simulink model "furuta_hybrid_model"  (R2026b)
settings: Solver=ode23t  StopTime=0.25  MaxStep=5.0000000000000002e-05  RelTol=1e-5  AbsTol=1e-8
model workspace (MAT data in the model file):
  cfg.sampleTime = 0.005
  cfg.energyGain = 100
  cfg.energyOffset = 0.04
  cfg.armCenterGain = 4
  cfg.armDampingGain = 3
  cfg.accelerationLimit = 25
  cfg.kickAcceleration = 3
  cfg.kickRate = 0.03
  cfg.signSlope = 8
  cfg.voltageLimit = 12
  cfg.captureAngle = 0.314159265359
  cfg.captureRate = 3
  cfg.captureArmRate = 3
  cfg.captureVoltage = 10
  cfg.releaseAngle = 0.610865238198
  cfg.releaseRate = 6
  cfg.armLimit = 3.14159265359
  cfg.speedLimit = 20
  disableTime = 100
  drive.voltageLimit = 12
  drive.resistance = 6.00258223899
  drive.backEmfOutput = 0.535780000531
  drive.torqueConstantOutput = 0.15
  drive.gearRatioSigned = -35.0048
  drive.gearRatio = 35.0048
  drive.motorShaftDamping = 4.08e-09
  drive.armatureInductance = 1.2003374e-05
  drive.gearEfficiency = 0.74571885855
  drive.speedGain = 1.74515107433
  drive.timeConstant = 0.200035574902
  drive.viscousDamping = 4.999370974e-06
  drive.reflectedInertia = 0.0028643583489
  drive.backEmfMotor = 0.0153059009202
  drive.torqueConstantMotor = 0.0057463031303
  drive.bridgeDrop = 2.55
  drive.pwmFrequency = 1000
  enableTime = 0
  furutaCoverImages.system = [242 242 242 242 242 242 242 242 242 242 242 242 ... (162435 elements, 221x245x3)]
  furutaCoverImages.bridge = [255 255 255 255 255 255 255 255 255 255 255 255 ... (561330 elements, 378x495x3)]
  furutaCoverImages.motor = [255 255 255 255 255 255 255 255 255 255 255 255 ... (578340 elements, 378x510x3)]
  furutaCoverImages.plant = [242 242 242 242 242 242 242 242 242 242 242 242 ... (57240 elements, 106x180x3)]
  initialState = [0; 3.14159265359; 0; 0]
  p.source = 'Revised Inventor Assembly1.iam with two fixed aluminum profiles'
  p.units = 'm, kg, kg*m^2, rad, N*m'
  p.parts(1).name = 'Motor_1'
  p.parts(1).source = 'cad\originals\inventor-package\modern control\modern control\Motor.ipt'
  p.parts(1).group = 'base'
  p.parts(1).rotation = [0.999875892244  0.0157543679293  8.87132397872e-16; 0.0157543679293  -0.999875892244  6.0713824632e-16; 8.96587377177e-16  -5.93086685557e-16  -1]
  p.parts(1).translation = [-7.8496237288e-17; 0; 0.0574]
  p.parts(1).mass = 0.117533764135
  p.parts(1).com = [-2.51629547723e-06; 7.77686868846e-05; 0.0334585043492]
  p.parts(1).inertia = [4.21856071427e-05  1.61868677081e-09  -2.41973308628e-09; 1.61868677081e-09  4.21259722545e-05  3.40164241998e-07; -2.41973308628e-09  3.40164241998e-07  9.42409412023e-06]
  p.parts(1).mesh = 'Motor_1.stl'
  p.parts(2).name = 'motor_holder_1'
  p.parts(2).source = 'cad\originals\inventor-package\modern control\modern control\motor holder.ipt'
  p.parts(2).group = 'base'
  p.parts(2).rotation = [-0.999993667555  -0.0035587708406  -8.83740457218e-16; 0.0035587708406  -0.999993667555  -6.03187801199e-16; -8.81588253822e-16  -6.06329011316e-16  1]
  p.parts(2).translation = [7.47341876526e-05; 0.0209998670187; 0.0183]
  p.parts(2).mass = 0.00752339947436
  p.parts(2).com = [1.89560478822e-14; 0.00840615914464; -0.00851588759587]
  p.parts(2).inertia = [1.56089117939e-06  -1.79636877134e-18  1.13827387038e-18; -1.79636877134e-18  1.27680196487e-06  4.44884161923e-07; 1.13827387038e-18  4.44884161923e-07  1.17145571104e-06]
  p.parts(2).mesh = 'motor_holder_1.stl'
  p.parts(3).name = 'Assembly2_1'
  p.parts(3).source = 'cad\originals\inventor-package\modern control\modern control\Assembly2\Assembly2.iam'
  p.parts(3).group = 'arm'
  p.parts(3).rotation = [-9.59608079282e-17  1.42983226155e-16  -1; 1.46439076445e-15  1  2.58616733772e-16; 1  -1.46439076445e-15  -9.59608079283e-17]
  p.parts(3).translation = [-0.00424079872686; -0.00199057601285; -0.0717771991128]
  p.parts(3).mass = 0.0256607587457
  p.parts(3).com = [0.0543345548641; 0.00199067178848; -0.00669149901998]
  p.parts(3).inertia = [3.76240629517e-06  -1.16658650356e-10  -1.25869727666e-06; -1.16658650356e-10  5.41849992051e-06  3.32034498219e-10; -1.25869727666e-06  3.32034498219e-10  5.39265534854e-06]
  p.parts(3).mesh = 'Assembly2_1.stl'
  p.parts(4).name = 'ROTERY_ENCODER_step_2'
  p.parts(4).source = 'cad\originals\inventor-package\modern control\modern control\ROTERY ENCODER.step.ipt'
  p.parts(4).group = 'arm'
  p.parts(4).rotation = [5.71932904618e-15  1  2.07325677924e-15; -0.795351383406  -6.03439045467e-16  -0.606148642591; -0.606148642591  4.20921426938e-17  0.795351383406]
  p.parts(4).translation = [-0.018; -2.55922809462e-17; -0.039]
  p.parts(4).mass = 0.362581648921
  p.parts(4).com = [-3.98602565469e-16; 0.0180945301807; 0.000779270131729]
  p.parts(4).inertia = [9.157701239e-05  -1.56720918563e-18  2.88926272881e-18; -1.56720918563e-18  8.38373271596e-05  3.64758854276e-06; 2.88926272881e-18  3.64758854276e-06  7.6668005389e-05]
  p.parts(4).mesh = 'ROTERY_ENCODER_step_2.stl'
  p.parts(5).name = 'Rigid_6_to_8mm_Coupler_v2_1'
  p.parts(5).source = 'cad\originals\inventor-package\modern control\modern control\Rigid 6 to 8mm Coupler v2.ipt'
  p.parts(5).group = 'pendulum'
  p.parts(5).rotation = [-0.433622184098  -0.901094779398  -8.17687882476e-17; 0.901094779398  -0.433622184098  7.14846949846e-16; 5.86197929882e-15  -1.76721434744e-15  1]
  p.parts(5).translation = [-2.41474407893e-15; -1.09599775774e-17; 0.02625]
  p.parts(5).mass = 0.0357095656133
  p.parts(5).com = [-1.98550332535e-05; 2.70878322074e-05; 0.0107724521144]
  p.parts(5).inertia = [2.06992966619e-06  9.78879116594e-10  1.79332086501e-09; 9.78879116594e-10  2.06855206248e-06  -1.36111507296e-09; 1.79332086501e-09  -1.36111507296e-09  1.26378706719e-06]
  p.parts(5).mesh = 'Rigid_6_to_8mm_Coupler_v2_1.stl'
  p.parts(6).name = 'ALLEN_04_mm_1'
  p.parts(6).source = 'cad\originals\inventor-package\modern control\modern control\ALLEN_04_mm.ipt'
  p.parts(6).group = 'pendulum'
  p.parts(6).rotation = [0.000757859024793  1.05403301233e-16  -0.999999712825; 0.999999712825  -7.14827144333e-16  0.000757859024793; 6.89644623391e-16  -1  -9.88333481276e-17]
  p.parts(6).translation = [-2.37309758457e-15; 6.34916804045e-18; -1.47627052195e-15]
  p.parts(6).mass = 0.0150565820614
  p.parts(6).com = [0.0494427569154; -0.00223584435412; 1.34932518455e-14]
  p.parts(6).inertia = [5.4161309878e-07  -1.66420228208e-06  1.00445586425e-17; -1.66420228208e-06  2.17246551386e-05  3.8628621652e-18; 1.00445586425e-17  3.8628621652e-18  2.22332408906e-05]
  p.parts(6).mesh = 'ALLEN_04_mm_1.stl'
  p.parts(7).name = 'Fixed_Profile_1'
  p.parts(7).source = 'cad\originals\inventor-package\modern control\modern control\80-20 Extrude aliminium.ipt'
  p.parts(7).group = 'base'
  p.parts(7).rotation = [0.999993667555  -0.0035587708406  1.36629504654e-16; -0.0035587708406  -0.999993667555  5.88565631011e-16; 8.66857020854e-16  -5.03645213996e-16  -1]
  p.parts(7).translation = [0.00709604248558; 0.0269749176281; 0.0008]
  p.parts(7).mass = 0.0267862913598
  p.parts(7).com = [-7.28208192606e-15; 2.68579367816e-18; -0.055]
  p.parts(7).inertia = [2.73817590257e-05  4.79616346638e-22  4.07673894642e-21; 4.79616346638e-22  2.73817590257e-05  -2.03836947321e-21; 4.07673894642e-21  -2.03836947321e-21  7.44497142427e-07]
  p.parts(7).mesh = 'Aluminum_Profile.stl'
  p.parts(8).name = 'Fixed_Profile_2'
  p.parts(8).source = 'cad\originals\inventor-package\modern control\modern control\80-20 Extrude aliminium.ipt'
  p.parts(8).group = 'base'
  p.parts(8).rotation = [0.999993667555  -0.0035587708406  1.51422143009e-16; -0.0035587708406  -0.999993667555  6.05793970765e-16; 8.81588253822e-16  -5.20926088263e-16  -1]
  p.parts(8).translation = [-0.00490388152508; 0.0270176228782; 0.0008]
  p.parts(8).mass = 0.0267862913598
  p.parts(8).com = [-7.28208192606e-15; 2.68579367816e-18; -0.055]
  p.parts(8).inertia = [2.73817590257e-05  4.79616346638e-22  4.07673894642e-21; 4.79616346638e-22  2.73817590257e-05  -2.03836947321e-21; 4.07673894642e-21  -2.03836947321e-21  7.44497142427e-07]
  p.parts(8).mesh = 'Aluminum_Profile.stl'
  p.arm.mass = 0.388242407666
  p.arm.com = [0.000250260496687; -0.000441127145441; -0.0369963448943]
  p.arm.inertia = [9.97410213472e-05  -2.23798970723e-06  2.9775733695e-06; -2.23798970723e-06  0.000102156432709  6.95047544707e-06; 2.9775733695e-06  6.95047544707e-06  8.60466122022e-05]
  p.pendulum.mass = 0.0507661476747
  p.pendulum.com = [-9.17674754395e-20; 0.0146432301305; 0.0267051946826]
  p.pendulum.inertia = [6.30406859376e-05  -4.54995494348e-08  2.13360006768e-08; -4.54995494348e-08  1.54268096381e-05  1.98932586949e-05; 2.13360006768e-08  1.98932586949e-05  4.89101053571e-05]
  p.hingeTranslation = [0.06925; -1.17961196366e-16; -0.039]
  p.hingeRotation = [3.29834787793e-18  0  -1; 1  0  -3.29834787793e-18; 0  -1  0]
  p.cadPendulumAngle = -1.57003840503
  p.armInertia = 0.00295050482616
  p.pendulumMass = 0.0507661476747
  p.pendulumCOMArmZero = [-0.0267051946826; -1.79850497651e-19; -0.0146432301305]
  p.pendulumInertiaArmZero = [4.89101053571e-05  -2.13360006768e-08  1.98932586949e-05; -2.13360006768e-08  6.30406859376e-05  4.54995494348e-08; 1.98932586949e-05  4.54995494348e-08  1.54268096381e-05]
  p.gravity = 9.81
  p.armDamping = 0.00010999945762
  p.pendulumDamping = 2.40372219881e-05
  p.initialState = [0; 3.24159265359; 0; 0]
  p.assumptions = {'Assembly2 is a rigid arm-mounted group despite its two unresolved source mates.'; 'ROTERY ENCODER.step:1 is excluded as an unmounted reference occurrence.'; 'The second encoder body is fixed to the arm; internal encoder rotor inertia is unavailable.'; 'Rigid coupler plus Allen key form the pendulum group.'; 'Rotor inertia and friction default to zero pending identification.'; 'The two grounded aluminum profiles and the motor holder are fixed to the world frame. Contact with moving bodies is not modeled.'; 'The assembly is physically rotated 180 degrees about its local X axis. Gravity remains world-down. Pendulum angle zero is physical upright.'}
  p.cadArmAngle = 2.25254684037
  p.mountRotation = [1  0  0; 0  -1  0; 0  0  -1]
undefined symbols (not defined in the file): X, Y, Z
libraries: sm_lib x23, nesl_utility x13, fl_lib x8, ee_lib x3
(part 1 of 2)
settings Model: Creator=yousef gharib  LastModifiedBy=yousef gharib
settings SolverCC: ZeroCrossAlgorithm=Adaptive
settings ModelReferenceCC: ModelReferenceMinAlgLoopOccurrences=on
settings SimscapeCC: SimscapeNominalValues="[{\"value\":\"1\",\"unit\":\"A\"},{\"value\":\"1\",\"unit\":\"bar\"},{\"value\":\"1\",\"unit\":\"cm^2\"},{\"value\":\"1\",\"unit\":\"cm^3/s\"},{\"value\":\"1\",\"unit\":\"kJ/kg\"},{\"value\":\"1\",\"unit\":\"kW\"},{\"value\":\"1\",\"unit\":\"l\"},{\"value\":\"1\",\"unit\":\"N\"},{\"value\":\"1\",\"unit\":\"N*m\"},{\"value\":\"1\",\"unit\":\"V\"},{\"value\":\"0.001\",\"unit\":\"Wb\"}]"  SimscapeUseEnergyAccounting=off

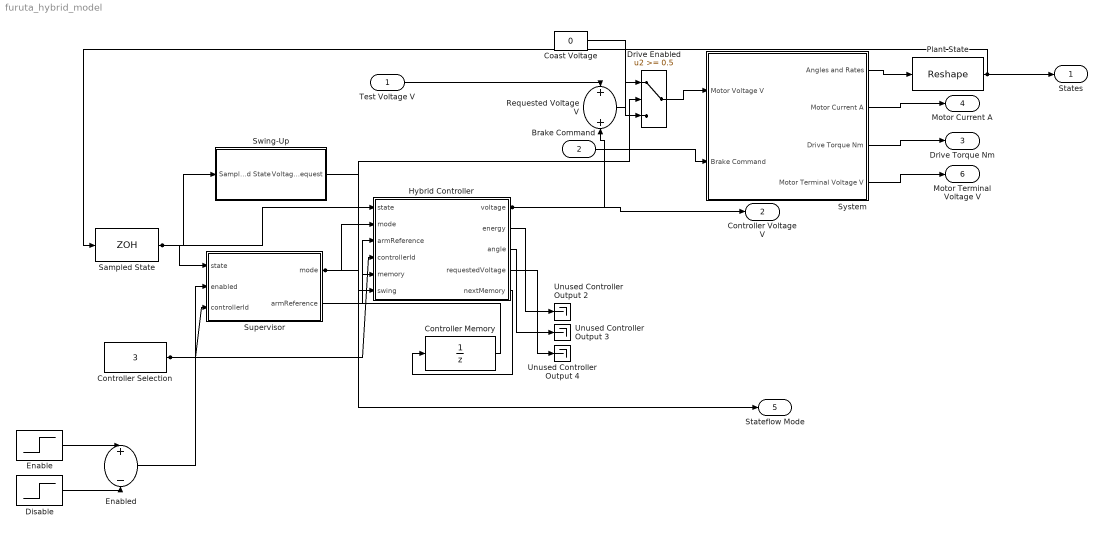
== system furuta_hybrid_model ==
  Test Voltage V : Inport
  Brake Command : Inport  Port=2
  Coast Voltage : Constant  Value=0
  Controller Memory : UnitDelay  InitialCondition=[0;0;0;-1;0]  SampleTime=cfg.sampleTime
  Controller Selection : Constant  Value=3  SampleTime=cfg.sampleTime
      settings: AttributesFormatString=|
      | 1 = PID/PD
      | 2 = Pole placement
      | 3 = LQR
  Disable : Step  Time=disableTime  SampleTime=cfg.sampleTime
  Drive Enabled : Switch  Threshold=0.5  SaturateOnIntegerOverflow=off  InputSameDT=off
  Enable : Step  Time=enableTime  SampleTime=cfg.sampleTime
  Enabled : Sum  Inputs=+-
  Hybrid Controller : MATLAB Function  TreatAsAtomicUnit=on
  Plant State : Reshape  OutputDimensionality=Column vector (2-D)
  Requested Voltage V : Sum
  Sampled State : ZeroOrderHold  SampleTime=cfg.sampleTime
  Supervisor : Stateflow chart  TreatAsAtomicUnit=on
  Swing-Up : Subsystem
  System : Subsystem
      mask help: Furuta pendulum with switching L298N drive and CAD plant.
      settings: OpenFcn=open_system(gcb,'force')
      mask Display:
      | covers = getVariable(get_param(bdroot(gcb),'ModelWorkspace'),'furutaCoverImages');
      | image(covers.system,[0 0 1 1]);
      | color('black');
      | port_label('input',1,'Command');
      | port_label('input',2,'Brake');
      | port_label('output',1,'States');
      | port_label('output',2,'Current');
      | port_label('output',3,'Torque');
      | port_label('output',4,'Voltage');
  Unused Controller Output 2 : Terminator
  Unused Controller Output 3 : Terminator
  Unused Controller Output 4 : Terminator
  States : Outport
  Controller Voltage V : Outport  Port=2
  Drive Torque Nm : Outport  Port=3
  Motor Current A : Outport  Port=4
  Stateflow Mode : Outport  Port=5
  Motor Terminal Voltage V : Outport  Port=6
  wires:
  Sampled State/1 -> Supervisor/1(state), Hybrid Controller/1(state), Swing-Up/1(Sampled State)
  Enable/1 -> Enabled/1
  Disable/1 -> Enabled/2
  Enabled/1 -> Supervisor/2(enabled)
  Controller Selection/1 -> Supervisor/3(controllerId), Hybrid Controller/4(controllerId)
  Test Voltage V/1 -> Requested Voltage V/1
  Hybrid Controller/1(voltage) -> Requested Voltage V/2, Controller Voltage V/1
  Brake Command/1 -> System/2(Brake Command)
  System/1(Angles and Rates) -> Plant State/1
  System/2(Motor Current A) -> Motor Current A/1
  System/3(Drive Torque Nm) -> Drive Torque Nm/1
  System/4(Motor Terminal Voltage V) -> Motor Terminal Voltage V/1
  Plant State/1 -> States/1, Sampled State/1
  Supervisor/1(mode) -> Hybrid Controller/2(mode), Stateflow Mode/1, Drive Enabled/2
  Supervisor/2(armReference) -> Hybrid Controller/3(armReference)
  Controller Memory/1 -> Hybrid Controller/5(memory)
  Swing-Up/1(Voltage Energy and Request) -> Hybrid Controller/6(swing)
  Hybrid Controller/5(nextMemory) -> Controller Memory/1
  Requested Voltage V/1 -> Drive Enabled/1
  Coast Voltage/1 -> Drive Enabled/3
  Drive Enabled/1 -> System/1(Motor Voltage V)
  Hybrid Controller/2(energy) -> Unused Controller Output 2/1
  Hybrid Controller/3(angle) -> Unused Controller Output 3/1
  Hybrid Controller/4(requestedVoltage) -> Unused Controller Output 4/1

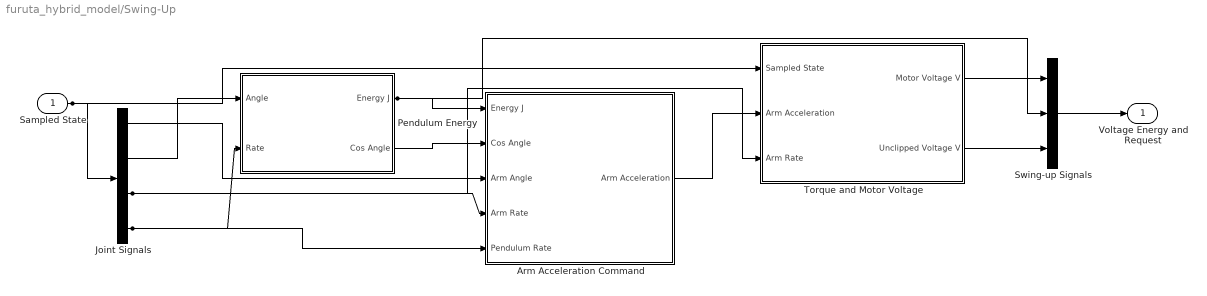
== system furuta_hybrid_model/Swing-Up ==
  Sampled State : Inport
  Arm Acceleration Command : Subsystem
  Joint Signals : Demux
  Pendulum Energy : Subsystem
  Swing-up Signals : Mux  Inputs=3
  Torque and Motor Voltage : Subsystem
  Voltage Energy and Request : Outport
  wires:
  Sampled State/1 -> Joint Signals/1, Torque and Motor Voltage/1(Sampled State)
  Swing-up Signals/1 -> Voltage Energy and Request/1
  Joint Signals/2 -> Pendulum Energy/1(Angle)
  Joint Signals/4 -> Pendulum Energy/2(Rate), Arm Acceleration Command/5(Pendulum Rate)
  Pendulum Energy/1(Energy J) -> Arm Acceleration Command/1(Energy J), Swing-up Signals/2
  Pendulum Energy/2(Cos Angle) -> Arm Acceleration Command/2(Cos Angle)
  Joint Signals/1 -> Arm Acceleration Command/3(Arm Angle)
  Joint Signals/3 -> Arm Acceleration Command/4(Arm Rate), Torque and Motor Voltage/3(Arm Rate)
  Arm Acceleration Command/1(Arm Acceleration) -> Torque and Motor Voltage/2(Arm Acceleration)
  Torque and Motor Voltage/1(Motor Voltage V) -> Swing-up Signals/1
  Torque and Motor Voltage/2(Unclipped Voltage V) -> Swing-up Signals/3

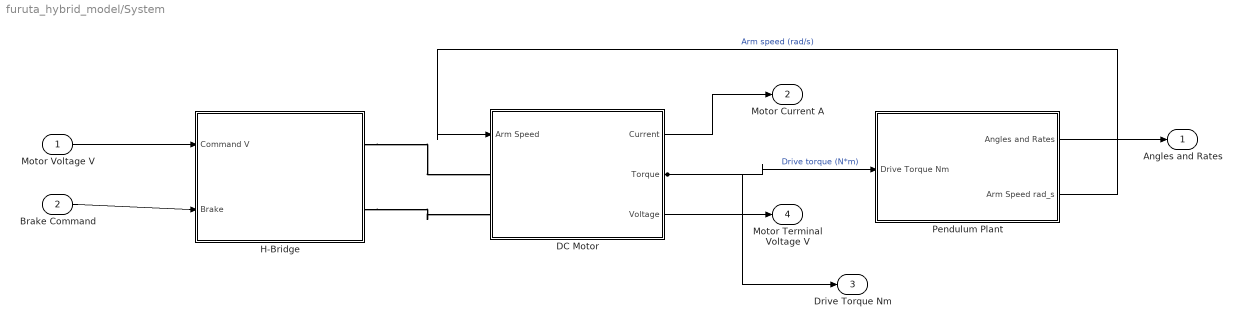
== system furuta_hybrid_model/System ==
  Motor Voltage V : Inport
  Brake Command : Inport  Port=2
  DC Motor : Subsystem
      mask help: GA25-370 geared motor and sensors. Photo from Most Electronics.
      settings: OpenFcn=open_system(gcb,'force')
      mask Display:
      | covers = getVariable(get_param(bdroot(gcb),'ModelWorkspace'),'furutaCoverImages');
      | image(covers.motor,[0 0 1 1]);
      | color('black');
      | port_label('input',1,'Arm Speed');
      | port_label('output',1,'Current');
      | port_label('output',2,'Torque');
      | port_label('output',3,'Voltage');
      | port_label('lconn',1,'+');
      | port_label('lconn',2,'-');
  H-Bridge : Subsystem
      mask help: L298N bridge and PWM logic. Photo from Addicore.
      settings: OpenFcn=open_system(gcb,'force')
      mask Display:
      | covers = getVariable(get_param(bdroot(gcb),'ModelWorkspace'),'furutaCoverImages');
      | image(covers.bridge,[0 0 1 1]);
      | color('black');
      | port_label('input',1,'Command');
      | port_label('input',2,'Brake');
      | port_label('rconn',1,'+');
      | port_label('rconn',2,'-');
  Pendulum Plant : Subsystem
      mask help: CAD-derived pendulum and arm mechanics.
      settings: OpenFcn=open_system(gcb,'force')
      mask Display:
      | covers = getVariable(get_param(bdroot(gcb),'ModelWorkspace'),'furutaCoverImages');
      | image(covers.plant,[0 0 1 1]);
      | color('black');
      | port_label('input',1,'Torque');
      | port_label('output',1,'States');
      | port_label('output',2,'Arm Speed');
  Angles and Rates : Outport
  Motor Current A : Outport  Port=2
  Drive Torque Nm : Outport  Port=3
  Motor Terminal Voltage V : Outport  Port=4
  wires:
  Pendulum Plant/2(Arm Speed rad_s) -> DC Motor/1(Arm Speed)  "Arm speed (rad/s)"
  DC Motor/3(Voltage) -> Motor Terminal Voltage V/1
  DC Motor/2(Torque) -> Drive Torque Nm/1, Pendulum Plant/1(Drive Torque Nm)  "Drive torque (N*m)"
  DC Motor/1(Current) -> Motor Current A/1
  Pendulum Plant/1(Angles and Rates) -> Angles and Rates/1
  Brake Command/1 -> H-Bridge/2(Brake)
  Motor Voltage V/1 -> H-Bridge/1(Command V)
  connections:
  H-Bridge/RConn2 -- DC Motor/LConn2
  H-Bridge/RConn1 -- DC Motor/LConn1

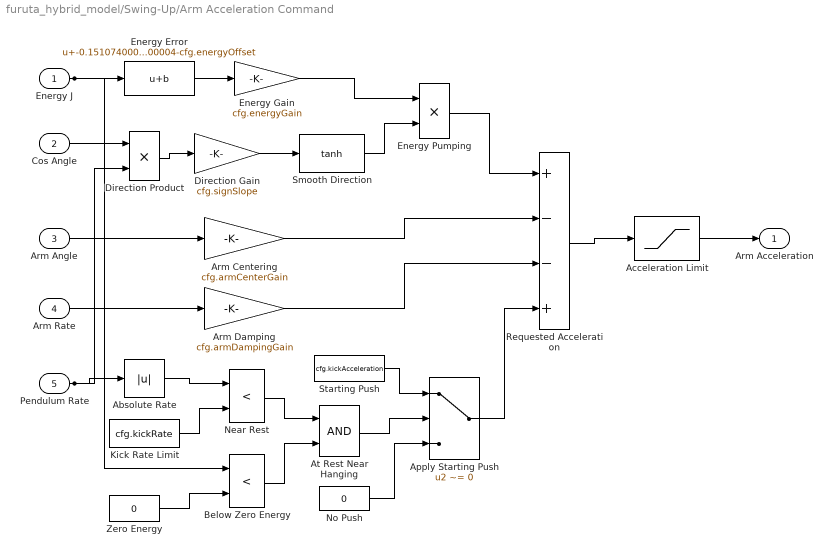
== system furuta_hybrid_model/Swing-Up/Arm Acceleration Command ==
  Energy J : Inport
  Cos Angle : Inport  Port=2
  Arm Angle : Inport  Port=3
  Arm Rate : Inport  Port=4
  Pendulum Rate : Inport  Port=5
  Absolute Rate : Abs  SaturateOnIntegerOverflow=off
  Acceleration Limit : Saturate  UpperLimit=cfg.accelerationLimit  LowerLimit=-cfg.accelerationLimit
  Apply Starting Push : Switch  Criteria=u2 ~= 0  SaturateOnIntegerOverflow=off  InputSameDT=off
  Arm Centering : Gain  Gain=cfg.armCenterGain
  Arm Damping : Gain  Gain=cfg.armDampingGain
  At Rest Near Hanging : Logic  AllPortsSameDT=off  OutDataTypeStr=boolean
  Below Zero Energy : RelationalOperator  Operator=<  OutDataTypeStr=boolean  RndMeth=Simplest  InputSameDT=off
  Direction Gain : Gain  Gain=cfg.signSlope
  Direction Product : Product
  Energy Error : Bias  Bias=-0.15107400000000004-cfg.energyOffset  SaturateOnIntegerOverflow=off
  Energy Gain : Gain  Gain=cfg.energyGain
  Energy Pumping : Product
  Kick Rate Limit : Constant  Value=cfg.kickRate
  Near Rest : RelationalOperator  Operator=<  OutDataTypeStr=boolean  RndMeth=Simplest  InputSameDT=off
  No Push : Constant  Value=0
  Requested Acceleration : Sum  Inputs=+--+
  Smooth Direction : Trigonometry  Operator=tanh
  Starting Push : Constant  Value=cfg.kickAcceleration
  Zero Energy : Constant  Value=0
  Arm Acceleration : Outport
  wires:
  Energy J/1 -> Energy Error/1, Below Zero Energy/1
  Energy Error/1 -> Energy Gain/1
  Cos Angle/1 -> Direction Product/1
  Pendulum Rate/1 -> Direction Product/2, Absolute Rate/1
  Direction Product/1 -> Direction Gain/1
  Direction Gain/1 -> Smooth Direction/1
  Energy Gain/1 -> Energy Pumping/1
  Smooth Direction/1 -> Energy Pumping/2
  Arm Angle/1 -> Arm Centering/1
  Arm Rate/1 -> Arm Damping/1
  Absolute Rate/1 -> Near Rest/1
  Kick Rate Limit/1 -> Near Rest/2
  Zero Energy/1 -> Below Zero Energy/2
  Near Rest/1 -> At Rest Near Hanging/1
  Below Zero Energy/1 -> At Rest Near Hanging/2
  Starting Push/1 -> Apply Starting Push/1
  At Rest Near Hanging/1 -> Apply Starting Push/2
  No Push/1 -> Apply Starting Push/3
  Energy Pumping/1 -> Requested Acceleration/1
  Arm Centering/1 -> Requested Acceleration/2
  Arm Damping/1 -> Requested Acceleration/3
  Apply Starting Push/1 -> Requested Acceleration/4
  Requested Acceleration/1 -> Acceleration Limit/1
  Acceleration Limit/1 -> Arm Acceleration/1

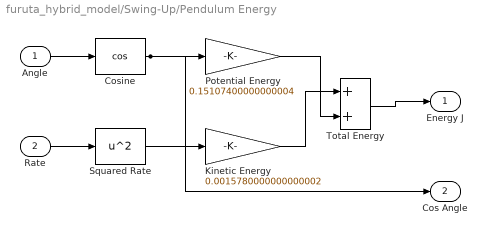
== system furuta_hybrid_model/Swing-Up/Pendulum Energy ==
  Angle : Inport
  Rate : Inport  Port=2
  Cosine : Trigonometry  Operator=cos
  Kinetic Energy : Gain  Gain=0.0015780000000000002
  Potential Energy : Gain  Gain=0.15107400000000004
  Squared Rate : Math  Operator=square
  Total Energy : Sum
  Energy J : Outport
  Cos Angle : Outport  Port=2
  wires:
  Angle/1 -> Cosine/1
  Rate/1 -> Squared Rate/1
  Cosine/1 -> Potential Energy/1, Cos Angle/1
  Squared Rate/1 -> Kinetic Energy/1
  Kinetic Energy/1 -> Total Energy/1
  Potential Energy/1 -> Total Energy/2
  Total Energy/1 -> Energy J/1

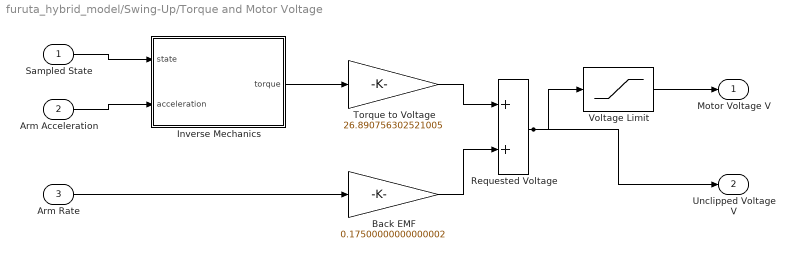
== system furuta_hybrid_model/Swing-Up/Torque and Motor Voltage ==
  Sampled State : Inport
  Arm Acceleration : Inport  Port=2
  Arm Rate : Inport  Port=3
  Back EMF : Gain  Gain=0.17500000000000002
  Inverse Mechanics : MATLAB Function  TreatAsAtomicUnit=on
  Requested Voltage : Sum
  Torque to Voltage : Gain  Gain=26.890756302521005
  Voltage Limit : Saturate  UpperLimit=cfg.voltageLimit  LowerLimit=-cfg.voltageLimit
  Motor Voltage V : Outport
  Unclipped Voltage V : Outport  Port=2
  wires:
  Arm Rate/1 -> Back EMF/1
  Torque to Voltage/1 -> Requested Voltage/1
  Back EMF/1 -> Requested Voltage/2
  Requested Voltage/1 -> Voltage Limit/1, Unclipped Voltage V/1
  Voltage Limit/1 -> Motor Voltage V/1
  Sampled State/1 -> Inverse Mechanics/1(state)
  Arm Acceleration/1 -> Inverse Mechanics/2(acceleration)
  Inverse Mechanics/1(torque) -> Torque to Voltage/1

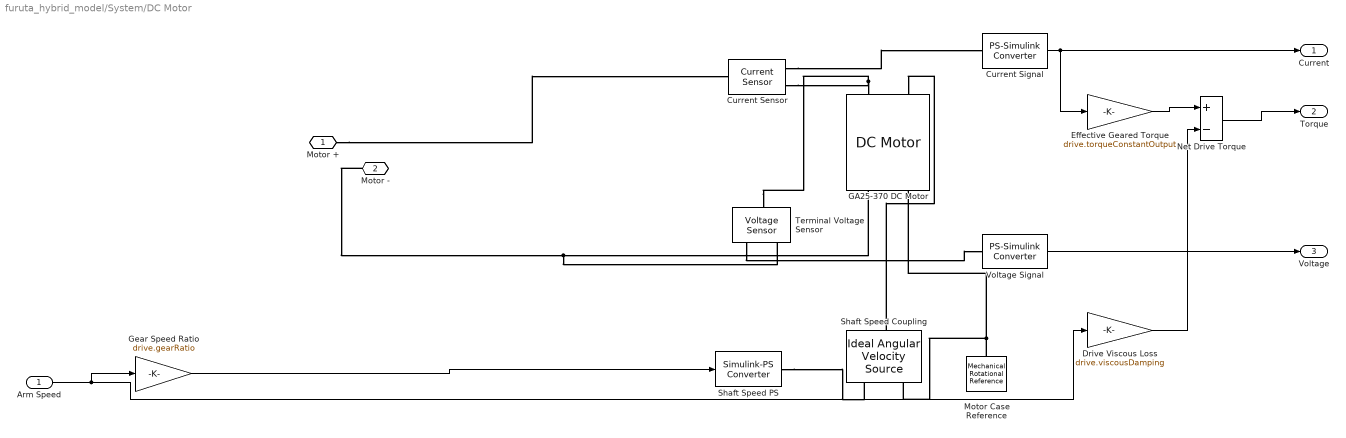
== system furuta_hybrid_model/System/DC Motor ==
  Arm Speed : Inport
  Current Sensor : fl_lib/Electrical/Electrical Sensors/Current Sensor
  Current Signal : nesl_utility/PS-Simulink Converter  PhysicalDomain=network_engine_domain  SubClassName=ps_output  LeftPortType=input  RightPortType=output  PseudoPeriodic=off  Frequencies=[]  VectorFormat=inherit  Unit=A  AffineConversion=off
  Drive Viscous Loss : Gain  Gain=drive.viscousDamping
  Effective Geared Torque : Gain  Gain=drive.torqueConstantOutput
  GA25-370 DC Motor : ee_lib/Electromechanical/Brushed Motors/DC Motor  field_option=ee.enum.field_option.pm  Rf=100 Ohm  Lf=1 H  Laf=0.15 H  If0=0 A  parameterization=ee.enum.dcparam_option.circuit_param  Ra=drive.resistance Ohm  La=drive.armatureInductance H  emf_or_torque=ee.enum.emf_or_torque.kv  Kv=drive.backEmfMotor V/(rad/s)  Ki=6.876e-4 N*m/A  T_stall=0.24e-3 N*m  w_max=19100 rpm  w_rated=15000 rpm  P_rated=0.08 W  V_rated=1.5 V  lam_param=ee.enum.lam_param.damping  i_noload=0 A  V_i_noload=1.5 V  J=drive.reflectedInertia/drive.gearRatio^2 kg*m^2  lam=0 N*m*s/rad  speed0=0 rpm  alpha=3.93e-3 1/K  Tmeas=25 degC  thermal_mass=100 J/K  initial_temperature=25 degC
  Gear Speed Ratio : Gain  Gain=drive.gearRatio
  Motor Case Reference : fl_lib/Mechanical/Rotational Elements/Mechanical Rotational Reference
  Net Drive Torque : Sum  Inputs=+-
  Shaft Speed Coupling : fl_lib/Mechanical/Mechanical Sources/Ideal Angular Velocity Source
  Shaft Speed PS : nesl_utility/Simulink-PS Converter  PhysicalDomain=network_engine_domain  SubClassName=ps_input  LeftPortType=input  RightPortType=output  PseudoPeriodic=off  Frequencies=[]  NoiseDistribution=none  NoiseParameters=[]  Unit=rad/s  AffineConversion=off  FilteringAndDerivatives=zero  SimscapeFilterOrder=1  InputFilterTimeConstant=0.001  UdotUserProvided=0
  Terminal Voltage Sensor : fl_lib/Electrical/Electrical Sensors/Voltage Sensor
  Voltage Signal : nesl_utility/PS-Simulink Converter  PhysicalDomain=network_engine_domain  SubClassName=ps_output  LeftPortType=input  RightPortType=output  PseudoPeriodic=off  Frequencies=[]  VectorFormat=inherit  Unit=V  AffineConversion=off
  Motor + : PMIOPort  Side=Left
  Motor - : PMIOPort  Port=2  Side=Left
  Current : Outport
  Torque : Outport  Port=2
  Voltage : Outport  Port=3
  wires:
  Voltage Signal/1 -> Voltage/1
  Gear Speed Ratio/1 -> Shaft Speed PS/1
  Net Drive Torque/1 -> Torque/1
  Effective Geared Torque/1 -> Net Drive Torque/1
  Arm Speed/1 -> Drive Viscous Loss/1, Gear Speed Ratio/1
  Current Signal/1 -> Effective Geared Torque/1, Current/1
  Drive Viscous Loss/1 -> Net Drive Torque/2
  connections:
  Motor +/RConn1 -- Current Sensor/LConn1
  Shaft Speed PS/RConn1 -- Shaft Speed Coupling/RConn1
  Shaft Speed Coupling/RConn2 -- Motor Case Reference/LConn1 -- GA25-370 DC Motor/RConn2
  Terminal Voltage Sensor/RConn2 -- Motor -/RConn1 -- GA25-370 DC Motor/RConn1
  Current Sensor/RConn1 -- Current Signal/LConn1
  Shaft Speed Coupling/LConn1 -- GA25-370 DC Motor/LConn2
  Terminal Voltage Sensor/LConn1 -- Current Sensor/RConn2 -- GA25-370 DC Motor/LConn1
  Terminal Voltage Sensor/RConn1 -- Voltage Signal/LConn1

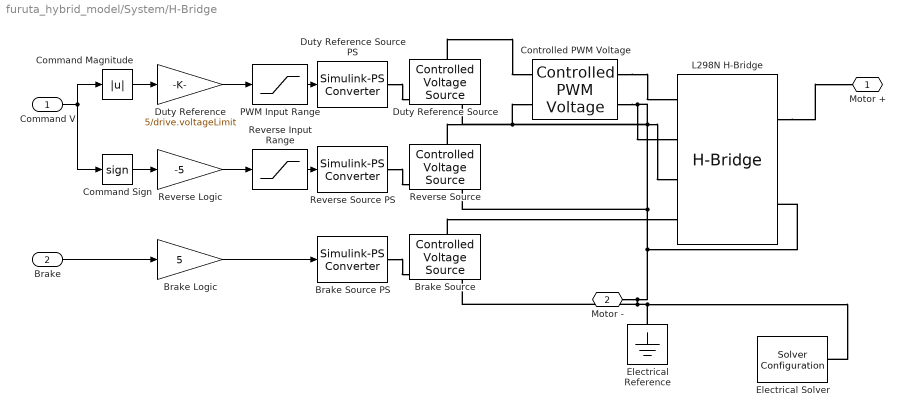
== system furuta_hybrid_model/System/H-Bridge ==
  Command V : Inport
  Brake : Inport  Port=2
  Brake Logic : Gain  Gain=5
  Brake Source : fl_lib/Electrical/Electrical Sources/Controlled Voltage Source
  Brake Source PS : nesl_utility/Simulink-PS Converter  PhysicalDomain=network_engine_domain  SubClassName=ps_input  LeftPortType=input  RightPortType=output  PseudoPeriodic=off  Frequencies=[]  NoiseDistribution=none  NoiseParameters=[]  Unit=V  AffineConversion=off  FilteringAndDerivatives=zero  SimscapeFilterOrder=1  InputFilterTimeConstant=0.001  UdotUserProvided=0
  Command Magnitude : Abs  SaturateOnIntegerOverflow=off
  Command Sign : Signum
  Controlled PWM Voltage : ee_lib/Integrated Circuits/Controlled PWM Voltage  F=drive.pwmFrequency Hz  TD=0 s  pulse_width_offset=0 s  pulse_min=0 s  pwm_or_av=ee.enum.pwm_or_av.pwm  event_type=ee.enum.ic.event.discrete  sample_time=1/(200*drive.pwmFrequency) s  Vmin=0 V  Vmax=5 V  Vm=5 V  u_min=0  u_max=1
  Duty Reference : Gain  Gain=5/drive.voltageLimit
  Duty Reference Source : fl_lib/Electrical/Electrical Sources/Controlled Voltage Source
  Duty Reference Source PS : nesl_utility/Simulink-PS Converter  PhysicalDomain=network_engine_domain  SubClassName=ps_input  LeftPortType=input  RightPortType=output  PseudoPeriodic=off  Frequencies=[]  NoiseDistribution=none  NoiseParameters=[]  Unit=V  AffineConversion=off  FilteringAndDerivatives=zero  SimscapeFilterOrder=1  InputFilterTimeConstant=0.001  UdotUserProvided=0
  Electrical Reference : fl_lib/Electrical/Electrical Elements/Electrical Reference
  Electrical Solver : nesl_utility/Solver Configuration  PhysicalDomain=network_engine_domain  SubClassName=solver  LeftPortType=input  RightPortType=generic  Tones=[]  Harmonics=[]  SimulateNoise=off  Profile=off  UseLocalSampling=off  EnableSwitchedLinearOptims=on  FrequencyDomain=off  UseCCode=off  RelTol=0.001  AbsTol=0.001  MinStep=1e-09  ToWorkspace=off  RevertToSquareIcSolve=off  NumHomotopyIterations=100  PhasorMode=off  PhasorModeNumHarmonics=1  ConsistencySolver=NEWTON_XTOL_AFTER_FTOL  CanonicalOrdering=CANONICAL  OptimizeIntermediates=OPTIMIZED  MulticoreSolverChoice=BACKWARD_EULER  IndexReductionMethod=DerivativeReplacement  DoDC=off  ResidualTolerance=1e-09  ConsistencyTolSource=GLOBAL  ConsistencyAbsTol=0.001  ConsistencyRelTol=0.001  ConsistencyTolFactor=0.001  UseLocalSolver=on  LocalSolverChoice=NE_BACKWARD_EULER_ADVANCER  ResolveIndetEquations=on  FunctionEvalNumThread=1  LocalSolverSampleTime=1/(200*drive.pwmFrequency)  DoFixedCost=off  MaxNonlinIter=3  MaxModeIter=2  ComputeImpulses=off  ImpulseIterations=2  LinearAlgebra=auto  LinearAlgebraNumThread=0  EquationFormulation=NE_TIME_EF  DelaysMemoryBudget=1024  AutomaticFiltering=on  FilteringTimeConstant=0.001  PartitionStorageMethod=AS_NEEDED  PartitionMemoryBudget=1024  PartitionMethod=BALANCED  MultibodyUseLocalSolver=off  MultibodyLocalSolverChoice=ODE1  MultibodyLocalSolverSampleTime=0.001
  L298N H-Bridge : ee_lib/Semiconductors & Converters/Converters/H-Bridge  supply_ports=ee.enum.supply_ports.hidesupply  pwm_or_av=ee.enum.pwm_or_av.pwm  discontinuous=ee.enum.current_profile.continuous  freewheeling_mode=ee.enum.converters.freewheeling_mode.two_diodes  Rload=10 Ohm  Lload=1e-5 H  F=10 kHz  regenerative_braking_mode=ee.enum.converters.regenerative_braking_mode.depends_on_rev  Venable=2.5 V  Vmax=5.0 V  Vreverse=2.5 V  Vbrake=2.5 V  Vm=drive.voltageLimit-drive.bridgeDrop V  Ron=0.1 Ohm  Don=0.05 Ohm  Goff=1e-6 S  Tmeas=298.15 K  Ron2=0.1 Ohm  Don2=0.05 Ohm  Tmeas2=398.15 K  thermal_mass=100 J/K  initial_temperature=298.15 K
  PWM Input Range : Saturate  UpperLimit=5  LowerLimit=0
  Reverse Input Range : Saturate  UpperLimit=5  LowerLimit=0
  Reverse Logic : Gain  Gain=-5
  Reverse Source : fl_lib/Electrical/Electrical Sources/Controlled Voltage Source
  Reverse Source PS : nesl_utility/Simulink-PS Converter  PhysicalDomain=network_engine_domain  SubClassName=ps_input  LeftPortType=input  RightPortType=output  PseudoPeriodic=off  Frequencies=[]  NoiseDistribution=none  NoiseParameters=[]  Unit=V  AffineConversion=off  FilteringAndDerivatives=zero  SimscapeFilterOrder=1  InputFilterTimeConstant=0.001  UdotUserProvided=0
  Motor + : PMIOPort  Side=Right
  Motor - : PMIOPort  Port=2  Side=Right
  wires:
  Brake/1 -> Brake Logic/1
  Brake Logic/1 -> Brake Source PS/1
  Reverse Input Range/1 -> Reverse Source PS/1
  Reverse Logic/1 -> Reverse Input Range/1
  Command Sign/1 -> Reverse Logic/1
  PWM Input Range/1 -> Duty Reference Source PS/1
  Command Magnitude/1 -> Duty Reference/1
  Duty Reference/1 -> PWM Input Range/1
  Command V/1 -> Command Sign/1, Command Magnitude/1
  connections:
  Reverse Source PS/RConn1 -- Reverse Source/RConn1
  Reverse Source/LConn1 -- L298N H-Bridge/LConn3
  Brake Source PS/RConn1 -- Brake Source/RConn1
  Electrical Solver/RConn1 -- Brake Source/RConn2 -- Motor -/RConn1 -- L298N H-Bridge/RConn2 -- Reverse Source/RConn2 -- L298N H-Bridge/LConn2 -- Controlled PWM Voltage/RConn2 -- Controlled PWM Voltage/LConn2 -- Duty Reference Source/RConn2 -- Electrical Reference/LConn1
  L298N H-Bridge/RConn1 -- Motor +/RConn1
  Brake Source/LConn1 -- L298N H-Bridge/LConn4
  Duty Reference Source PS/RConn1 -- Duty Reference Source/RConn1
  Duty Reference Source/LConn1 -- Controlled PWM Voltage/LConn1
  Controlled PWM Voltage/RConn1 -- L298N H-Bridge/LConn1

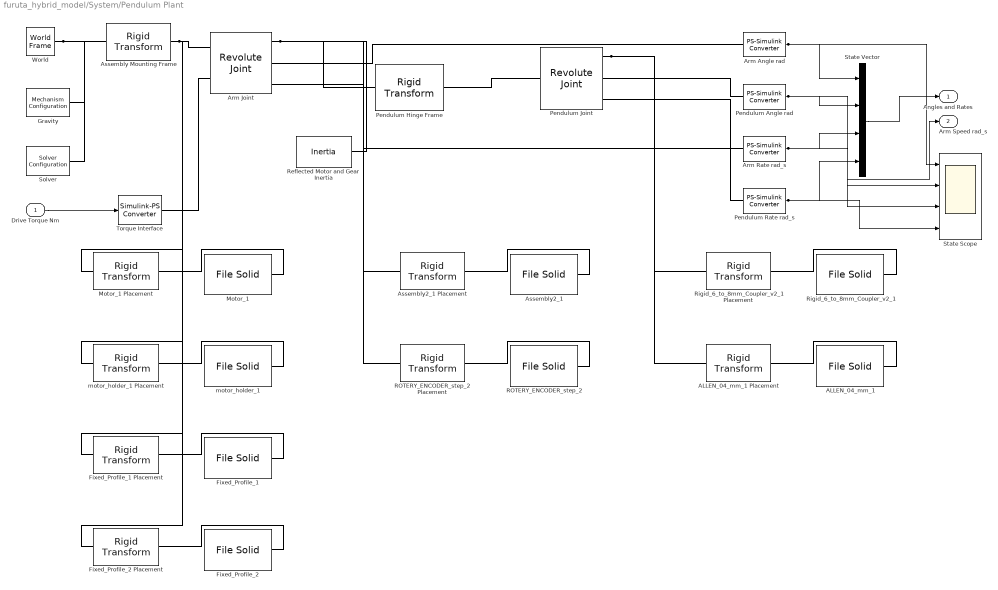
== system furuta_hybrid_model/System/Pendulum Plant ==
  Drive Torque Nm : Inport
  ALLEN_04_mm_1 : sm_lib/Body Elements/File Solid  ExtGeomFileName=D:\university new\Modern Control\project\cad\simscape-exports\ALLEN_04_mm_1.stl  UnitType=Custom  ExtGeomFileUnits=m  StepReaderType=HEX  ExportConvexHullGeometry=off  InertiaType=Custom  BasedOnType=DensityFromFile  Density=1000  DensityUnits=kg/m^3  Mass=0.015056582061423344  MassUnits=kg  CenterOfMass=[0.049442756915436939 -0.0022358443541156924 1.349325184547749e-14]  CenterOfMassUnits=m  MomentsOfInertia=[5.4161309878027966e-07 2.1724655138574078e-05 2.2233240890625076e-05]  MomentsOfInertiaUnits=kg*m^2  ProductsOfInertia=[3.8628621652012637e-18 1.0044558642473713e-17 -1.664202282079325e-06]  ProductsOfInertiaUnits=kg*m^2  GraphicType=FromGeometry  MarkerShape=Sphere  MarkerSize=10  GraphicVisPropType=SimpleVisualProperties  GraphicDiffuseColor=[0.5 0.5 0.5]  GraphicOpacity=1  GraphicSpecularColor=[0.5 0.5 0.5 1.0]  GraphicAmbientColor=[0.15 0.15 0.15 1.0]  GraphicEmissiveColor=[0.0 0.0 0.0 1.0]  GraphicShininess=75  DoExposeReferenceFrame=on  SerializedFrames=<Frames/>
  ALLEN_04_mm_1 Placement : sm_lib/Frames and Transforms/Rigid Transform  RotationMethod=RotationMatrix  FollAlignAxisA=+X  BaseAlignAxisA=+Y  FollAlignAxisB=+Y  BaseAlignAxisB=+Z  RotationStandardAxis=+Z  RotationAngle=0  RotationAngleUnits=deg  RotationArbitraryAxis=[0 0 1]  RotationSequenceAxes=FollowerAxes  RotationSequence=XYX  RotationSequenceAngles=[0 0 0]  RotationSequenceAnglesUnits=deg  RotationMatrix=p.parts(6).rotation  Quaternion=[1 0 0 0]  TranslationMethod=Cartesian  TranslationCartesianOffset=p.parts(6).translation  TranslationCartesianOffsetUnits=m  TranslationStandardAxis=+Z  TranslationStandardOffset=0  TranslationStandardOffsetUnits=m  TranslationROffset=0  TranslationROffsetUnits=m  TranslationThetaOffset=0  TranslationThetaOffsetUnits=deg  TranslationZOffset=0  TranslationZOffsetUnits=m
  Arm Angle rad : nesl_utility/PS-Simulink Converter  PhysicalDomain=network_engine_domain  SubClassName=ps_output  LeftPortType=input  RightPortType=output  PseudoPeriodic=off  Frequencies=[]  VectorFormat=inherit  Unit=rad  AffineConversion=off
  Arm Joint : sm_lib/Joints/Revolute Joint  JointMode=Normal  CompositeWrenchDir=FollowerOnBase  CompositeWrenchFrame=BaseFrame  SenseConstraintForce=off  SenseConstraintTorque=off  SenseTotalForce=off  SenseTotalTorque=off  PositionTargetSpecify=on  PositionTargetPriority=High  PositionTargetValue=initialState(1)  PositionTargetValueUnits=rad  VelocityTargetSpecify=on  VelocityTargetPriority=High  VelocityTargetValue=initialState(3)  VelocityTargetValueUnits=rad/s  EquilibriumPosition=0  EquilibriumPositionUnits=deg  SpringStiffness=0  SpringStiffnessUnits=N*m/deg  DampingCoefficient=p.armDamping  DampingCoefficientUnits=N*m/(rad/s)  LowerLimitSpecify=off  LowerLimitBound=-90  LowerLimitBoundUnits=deg  LowerLimitStiffness=1e4  LowerLimitStiffnessUnits=N*m/deg  LowerLimitDamping=10  LowerLimitDampingUnits=N*m/(deg/s)  LowerLimitTransitionRegionWidth=0.1  LowerLimitTransitionRegionWidthUnits=deg  UpperLimitSpecify=off  UpperLimitBound=90  UpperLimitBoundUnits=deg  UpperLimitStiffness=1e4  UpperLimitStiffnessUnits=N*m/deg  UpperLimitDamping=10  UpperLimitDampingUnits=N*m/(deg/s)  UpperLimitTransitionRegionWidth=0.1  UpperLimitTransitionRegionWidthUnits=deg  TorqueActuationMode=InputTorque  MotionActuationMode=ComputedMotion  SensePosition=on  SenseVelocity=on  SenseAcceleration=off  SenseTorqueForce=off  SenseLowerLimitTorqueForce=off  SenseUpperLimitTorqueForce=off
  Arm Rate rad_s : nesl_utility/PS-Simulink Converter  PhysicalDomain=network_engine_domain  SubClassName=ps_output  LeftPortType=input  RightPortType=output  PseudoPeriodic=off  Frequencies=[]  VectorFormat=inherit  Unit=rad/s  AffineConversion=off
  Assembly Mounting Frame : sm_lib/Frames and Transforms/Rigid Transform  RotationMethod=RotationMatrix  FollAlignAxisA=+X  BaseAlignAxisA=+Y  FollAlignAxisB=+Y  BaseAlignAxisB=+Z  RotationStandardAxis=+Z  RotationAngle=0  RotationAngleUnits=deg  RotationArbitraryAxis=[0 0 1]  RotationSequenceAxes=FollowerAxes  RotationSequence=XYX  RotationSequenceAngles=[0 0 0]  RotationSequenceAnglesUnits=deg  RotationMatrix=p.mountRotation  Quaternion=[1 0 0 0]  TranslationMethod=None  TranslationCartesianOffset=[0 0 0]  TranslationCartesianOffsetUnits=m  TranslationStandardAxis=+Z  TranslationStandardOffset=0  TranslationStandardOffsetUnits=m  TranslationROffset=0  TranslationROffsetUnits=m  TranslationThetaOffset=0  TranslationThetaOffsetUnits=deg  TranslationZOffset=0  TranslationZOffsetUnits=m
  Assembly2_1 : sm_lib/Body Elements/File Solid  ExtGeomFileName=D:\university new\Modern Control\project\cad\simscape-exports\Assembly2_1.stl  UnitType=Custom  ExtGeomFileUnits=m  StepReaderType=HEX  ExportConvexHullGeometry=off  InertiaType=Custom  BasedOnType=DensityFromFile  Density=1000  DensityUnits=kg/m^3  Mass=0.025660758745707356  MassUnits=kg  CenterOfMass=[0.054334554864073049 0.0019906717884835721 -0.0066914990199800559]  CenterOfMassUnits=m  MomentsOfInertia=[3.7624062951651073e-06 5.4184999205071335e-06 5.3926553485442469e-06]  MomentsOfInertiaUnits=kg*m^2  ProductsOfInertia=[3.3203449821934683e-10 -1.2586972766629928e-06 -1.1665865035581647e-10]  ProductsOfInertiaUnits=kg*m^2  GraphicType=FromGeometry  MarkerShape=Sphere  MarkerSize=10  GraphicVisPropType=SimpleVisualProperties  GraphicDiffuseColor=[0.5 0.5 0.5]  GraphicOpacity=1  GraphicSpecularColor=[0.5 0.5 0.5 1.0]  GraphicAmbientColor=[0.15 0.15 0.15 1.0]  GraphicEmissiveColor=[0.0 0.0 0.0 1.0]  GraphicShininess=75  DoExposeReferenceFrame=on  SerializedFrames=<Frames/>
  Assembly2_1 Placement : sm_lib/Frames and Transforms/Rigid Transform  RotationMethod=RotationMatrix  FollAlignAxisA=+X  BaseAlignAxisA=+Y  FollAlignAxisB=+Y  BaseAlignAxisB=+Z  RotationStandardAxis=+Z  RotationAngle=0  RotationAngleUnits=deg  RotationArbitraryAxis=[0 0 1]  RotationSequenceAxes=FollowerAxes  RotationSequence=XYX  RotationSequenceAngles=[0 0 0]  RotationSequenceAnglesUnits=deg  RotationMatrix=p.parts(3).rotation  Quaternion=[1 0 0 0]  TranslationMethod=Cartesian  TranslationCartesianOffset=p.parts(3).translation  TranslationCartesianOffsetUnits=m  TranslationStandardAxis=+Z  TranslationStandardOffset=0  TranslationStandardOffsetUnits=m  TranslationROffset=0  TranslationROffsetUnits=m  TranslationThetaOffset=0  TranslationThetaOffsetUnits=deg  TranslationZOffset=0  TranslationZOffsetUnits=m
  Fixed_Profile_1 : sm_lib/Body Elements/File Solid  ExtGeomFileName=D:\university new\Modern Control\project\cad\simscape-exports\Aluminum_Profile.stl  UnitType=Custom  ExtGeomFileUnits=m  StepReaderType=HEX  ExportConvexHullGeometry=off  InertiaType=Custom  BasedOnType=DensityFromFile  Density=1000  DensityUnits=kg/m^3  Mass=0.026786291359838666  MassUnits=kg  CenterOfMass=[-7.2820819260616346e-15 2.6857936781638681e-18 -0.054999999999999993]  CenterOfMassUnits=m  MomentsOfInertia=[2.7381759025687315e-05 2.7381759025747546e-05 7.4449714242688537e-07]  MomentsOfInertiaUnits=kg*m^2  ProductsOfInertia=[-2.0383694732117867e-21 4.0767389464230581e-21 4.7961634663754375e-22]  ProductsOfInertiaUnits=kg*m^2  GraphicType=FromGeometry  MarkerShape=Sphere  MarkerSize=10  GraphicVisPropType=SimpleVisualProperties  GraphicDiffuseColor=[0.5 0.5 0.5]  GraphicOpacity=1  GraphicSpecularColor=[0.5 0.5 0.5 1.0]  GraphicAmbientColor=[0.15 0.15 0.15 1.0]  GraphicEmissiveColor=[0.0 0.0 0.0 1.0]  GraphicShininess=75  DoExposeReferenceFrame=on  SerializedFrames=<Frames/>
  Fixed_Profile_1 Placement : sm_lib/Frames and Transforms/Rigid Transform  RotationMethod=RotationMatrix  FollAlignAxisA=+X  BaseAlignAxisA=+Y  FollAlignAxisB=+Y  BaseAlignAxisB=+Z  RotationStandardAxis=+Z  RotationAngle=0  RotationAngleUnits=deg  RotationArbitraryAxis=[0 0 1]  RotationSequenceAxes=FollowerAxes  RotationSequence=XYX  RotationSequenceAngles=[0 0 0]  RotationSequenceAnglesUnits=deg  RotationMatrix=p.parts(7).rotation  Quaternion=[1 0 0 0]  TranslationMethod=Cartesian  TranslationCartesianOffset=p.parts(7).translation  TranslationCartesianOffsetUnits=m  TranslationStandardAxis=+Z  TranslationStandardOffset=0  TranslationStandardOffsetUnits=m  TranslationROffset=0  TranslationROffsetUnits=m  TranslationThetaOffset=0  TranslationThetaOffsetUnits=deg  TranslationZOffset=0  TranslationZOffsetUnits=m
  Fixed_Profile_2 : sm_lib/Body Elements/File Solid  ExtGeomFileName=D:\university new\Modern Control\project\cad\simscape-exports\Aluminum_Profile.stl  UnitType=Custom  ExtGeomFileUnits=m  StepReaderType=HEX  ExportConvexHullGeometry=off  InertiaType=Custom  BasedOnType=DensityFromFile  Density=1000  DensityUnits=kg/m^3  Mass=0.026786291359838666  MassUnits=kg  CenterOfMass=[-7.2820819260616346e-15 2.6857936781638681e-18 -0.054999999999999993]  CenterOfMassUnits=m  MomentsOfInertia=[2.7381759025687315e-05 2.7381759025747546e-05 7.4449714242688537e-07]  MomentsOfInertiaUnits=kg*m^2  ProductsOfInertia=[-2.0383694732117867e-21 4.0767389464230581e-21 4.7961634663754375e-22]  ProductsOfInertiaUnits=kg*m^2  GraphicType=FromGeometry  MarkerShape=Sphere  MarkerSize=10  GraphicVisPropType=SimpleVisualProperties  GraphicDiffuseColor=[0.5 0.5 0.5]  GraphicOpacity=1  GraphicSpecularColor=[0.5 0.5 0.5 1.0]  GraphicAmbientColor=[0.15 0.15 0.15 1.0]  GraphicEmissiveColor=[0.0 0.0 0.0 1.0]  GraphicShininess=75  DoExposeReferenceFrame=on  SerializedFrames=<Frames/>
  Fixed_Profile_2 Placement : sm_lib/Frames and Transforms/Rigid Transform  RotationMethod=RotationMatrix  FollAlignAxisA=+X  BaseAlignAxisA=+Y  FollAlignAxisB=+Y  BaseAlignAxisB=+Z  RotationStandardAxis=+Z  RotationAngle=0  RotationAngleUnits=deg  RotationArbitraryAxis=[0 0 1]  RotationSequenceAxes=FollowerAxes  RotationSequence=XYX  RotationSequenceAngles=[0 0 0]  RotationSequenceAnglesUnits=deg  RotationMatrix=p.parts(8).rotation  Quaternion=[1 0 0 0]  TranslationMethod=Cartesian  TranslationCartesianOffset=p.parts(8).translation  TranslationCartesianOffsetUnits=m  TranslationStandardAxis=+Z  TranslationStandardOffset=0  TranslationStandardOffsetUnits=m  TranslationROffset=0  TranslationROffsetUnits=m  TranslationThetaOffset=0  TranslationThetaOffsetUnits=deg  TranslationZOffset=0  TranslationZOffsetUnits=m
  Gravity : sm_lib/Utilities/Mechanism Configuration  UniformGravity=Constant  GravityVector=[0 0 -p.gravity]  GravityVectorUnits=m/s^2  LinearizationDelta=0.001  JointModeTransitionNonlinearIterations=2
  Motor_1 : sm_lib/Body Elements/File Solid  ExtGeomFileName=D:\university new\Modern Control\project\cad\simscape-exports\Motor_1.stl  UnitType=Custom  ExtGeomFileUnits=m  StepReaderType=HEX  ExportConvexHullGeometry=off  InertiaType=Custom  BasedOnType=DensityFromFile  Density=1000  DensityUnits=kg/m^3  Mass=0.11753376413462681  MassUnits=kg  CenterOfMass=[-2.5162954772292185e-06 7.7768686884598968e-05 0.033458504349221832]  CenterOfMassUnits=m  MomentsOfInertia=[4.2185607142697659e-05 4.2125972254480369e-05 9.4240941202343113e-06]  MomentsOfInertiaUnits=kg*m^2  ProductsOfInertia=[3.4016424199841635e-07 -2.4197330862763226e-09 1.618686770812268e-09]  ProductsOfInertiaUnits=kg*m^2  GraphicType=FromGeometry  MarkerShape=Sphere  MarkerSize=10  GraphicVisPropType=SimpleVisualProperties  GraphicDiffuseColor=[0.5 0.5 0.5]  GraphicOpacity=1  GraphicSpecularColor=[0.5 0.5 0.5 1.0]  GraphicAmbientColor=[0.15 0.15 0.15 1.0]  GraphicEmissiveColor=[0.0 0.0 0.0 1.0]  GraphicShininess=75  DoExposeReferenceFrame=on  SerializedFrames=<Frames/>
  Motor_1 Placement : sm_lib/Frames and Transforms/Rigid Transform  RotationMethod=RotationMatrix  FollAlignAxisA=+X  BaseAlignAxisA=+Y  FollAlignAxisB=+Y  BaseAlignAxisB=+Z  RotationStandardAxis=+Z  RotationAngle=0  RotationAngleUnits=deg  RotationArbitraryAxis=[0 0 1]  RotationSequenceAxes=FollowerAxes  RotationSequence=XYX  RotationSequenceAngles=[0 0 0]  RotationSequenceAnglesUnits=deg  RotationMatrix=p.parts(1).rotation  Quaternion=[1 0 0 0]  TranslationMethod=Cartesian  TranslationCartesianOffset=p.parts(1).translation  TranslationCartesianOffsetUnits=m  TranslationStandardAxis=+Z  TranslationStandardOffset=0  TranslationStandardOffsetUnits=m  TranslationROffset=0  TranslationROffsetUnits=m  TranslationThetaOffset=0  TranslationThetaOffsetUnits=deg  TranslationZOffset=0  TranslationZOffsetUnits=m
  Pendulum Angle rad : nesl_utility/PS-Simulink Converter  PhysicalDomain=network_engine_domain  SubClassName=ps_output  LeftPortType=input  RightPortType=output  PseudoPeriodic=off  Frequencies=[]  VectorFormat=inherit  Unit=rad  AffineConversion=off
  Pendulum Hinge Frame : sm_lib/Frames and Transforms/Rigid Transform  RotationMethod=RotationMatrix  FollAlignAxisA=+X  BaseAlignAxisA=+Y  FollAlignAxisB=+Y  BaseAlignAxisB=+Z  RotationStandardAxis=+Z  RotationAngle=0  RotationAngleUnits=deg  RotationArbitraryAxis=[0 0 1]  RotationSequenceAxes=FollowerAxes  RotationSequence=XYX  RotationSequenceAngles=[0 0 0]  RotationSequenceAnglesUnits=deg  RotationMatrix=p.hingeRotation  Quaternion=[1 0 0 0]  TranslationMethod=Cartesian  TranslationCartesianOffset=p.hingeTranslation  TranslationCartesianOffsetUnits=m  TranslationStandardAxis=+Z  TranslationStandardOffset=0  TranslationStandardOffsetUnits=m  TranslationROffset=0  TranslationROffsetUnits=m  TranslationThetaOffset=0  TranslationThetaOffsetUnits=deg  TranslationZOffset=0  TranslationZOffsetUnits=m
  Pendulum Joint : sm_lib/Joints/Revolute Joint  JointMode=Normal  CompositeWrenchDir=FollowerOnBase  CompositeWrenchFrame=BaseFrame  SenseConstraintForce=off  SenseConstraintTorque=off  SenseTotalForce=off  SenseTotalTorque=off  PositionTargetSpecify=on  PositionTargetPriority=High  PositionTargetValue=initialState(2)  PositionTargetValueUnits=rad  VelocityTargetSpecify=on  VelocityTargetPriority=High  VelocityTargetValue=initialState(4)  VelocityTargetValueUnits=rad/s  EquilibriumPosition=0  EquilibriumPositionUnits=deg  SpringStiffness=0  SpringStiffnessUnits=N*m/deg  DampingCoefficient=p.pendulumDamping  DampingCoefficientUnits=N*m/(rad/s)  LowerLimitSpecify=off  LowerLimitBound=-90  LowerLimitBoundUnits=deg  LowerLimitStiffness=1e4  LowerLimitStiffnessUnits=N*m/deg  LowerLimitDamping=10  LowerLimitDampingUnits=N*m/(deg/s)  LowerLimitTransitionRegionWidth=0.1  LowerLimitTransitionRegionWidthUnits=deg  UpperLimitSpecify=off  UpperLimitBound=90  UpperLimitBoundUnits=deg  UpperLimitStiffness=1e4  UpperLimitStiffnessUnits=N*m/deg  UpperLimitDamping=10  UpperLimitDampingUnits=N*m/(deg/s)  UpperLimitTransitionRegionWidth=0.1  UpperLimitTransitionRegionWidthUnits=deg  TorqueActuationMode=NoTorque  MotionActuationMode=ComputedMotion  SensePosition=on  SenseVelocity=on  SenseAcceleration=off  SenseTorqueForce=off  SenseLowerLimitTorqueForce=off  SenseUpperLimitTorqueForce=off
  Pendulum Rate rad_s : nesl_utility/PS-Simulink Converter  PhysicalDomain=network_engine_domain  SubClassName=ps_output  LeftPortType=input  RightPortType=output  PseudoPeriodic=off  Frequencies=[]  VectorFormat=inherit  Unit=rad/s  AffineConversion=off
  ROTERY_ENCODER_step_2 : sm_lib/Body Elements/File Solid  ExtGeomFileName=D:\university new\Modern Control\project\cad\simscape-exports\ROTERY_ENCODER_step_2.stl  UnitType=Custom  ExtGeomFileUnits=m  StepReaderType=HEX  ExportConvexHullGeometry=off  InertiaType=Custom  BasedOnType=DensityFromFile  Density=1000  DensityUnits=kg/m^3  Mass=0.36258164892070927  MassUnits=kg  CenterOfMass=[-3.9860256546864253e-16 0.018094530180718476 0.00077927013172852727]  CenterOfMassUnits=m  MomentsOfInertia=[9.1577012389985557e-05 8.3837327159576086e-05 7.6668005388956037e-05]  MomentsOfInertiaUnits=kg*m^2  ProductsOfInertia=[3.6475885427603122e-06 2.8892627288068479e-18 -1.5672091856309675e-18]  ProductsOfInertiaUnits=kg*m^2  GraphicType=FromGeometry  MarkerShape=Sphere  MarkerSize=10  GraphicVisPropType=SimpleVisualProperties  GraphicDiffuseColor=[0.5 0.5 0.5]  GraphicOpacity=1  GraphicSpecularColor=[0.5 0.5 0.5 1.0]  GraphicAmbientColor=[0.15 0.15 0.15 1.0]  GraphicEmissiveColor=[0.0 0.0 0.0 1.0]  GraphicShininess=75  DoExposeReferenceFrame=on  SerializedFrames=<Frames/>
  ROTERY_ENCODER_step_2 Placement : sm_lib/Frames and Transforms/Rigid Transform  RotationMethod=RotationMatrix  FollAlignAxisA=+X  BaseAlignAxisA=+Y  FollAlignAxisB=+Y  BaseAlignAxisB=+Z  RotationStandardAxis=+Z  RotationAngle=0  RotationAngleUnits=deg  RotationArbitraryAxis=[0 0 1]  RotationSequenceAxes=FollowerAxes  RotationSequence=XYX  RotationSequenceAngles=[0 0 0]  RotationSequenceAnglesUnits=deg  RotationMatrix=p.parts(4).rotation  Quaternion=[1 0 0 0]  TranslationMethod=Cartesian  TranslationCartesianOffset=p.parts(4).translation  TranslationCartesianOffsetUnits=m  TranslationStandardAxis=+Z  TranslationStandardOffset=0  TranslationStandardOffsetUnits=m  TranslationROffset=0  TranslationROffsetUnits=m  TranslationThetaOffset=0  TranslationThetaOffsetUnits=deg  TranslationZOffset=0  TranslationZOffsetUnits=m
  Reflected Motor and Gear Inertia : sm_lib/Body Elements/Inertia  InertiaType=Custom  Mass=0  MassUnits=kg  CenterOfMass=[0 0 0]  CenterOfMassUnits=m  MomentsOfInertia=drive.reflectedInertia*[0.5 0.5 1]  MomentsOfInertiaUnits=kg*m^2  ProductsOfInertia=[0 0 0]  ProductsOfInertiaUnits=kg*m^2  GraphicType=Marker  MarkerShape=Inertia  MarkerSize=20  GraphicVisPropType=SimpleVisualProperties  GraphicDiffuseColor=[0.5 0.5 0.5]  GraphicOpacity=1  GraphicSpecularColor=[0.5 0.5 0.5 1.0]  GraphicAmbientColor=[0.15 0.15 0.15 1.0]  GraphicEmissiveColor=[0.0 0.0 0.0 1.0]  GraphicShininess=75
  Rigid_6_to_8mm_Coupler_v2_1 : sm_lib/Body Elements/File Solid  ExtGeomFileName=D:\university new\Modern Control\project\cad\simscape-exports\Rigid_6_to_8mm_Coupler_v2_1.stl  UnitType=Custom  ExtGeomFileUnits=m  StepReaderType=HEX  ExportConvexHullGeometry=off  InertiaType=Custom  BasedOnType=DensityFromFile  Density=1000  DensityUnits=kg/m^3  Mass=0.035709565613316965  MassUnits=kg  CenterOfMass=[-1.9855033253483611e-05 2.7087832207430867e-05 0.010772452114430477]  CenterOfMassUnits=m  MomentsOfInertia=[2.0699296661938313e-06 2.0685520624845489e-06 1.2637870671925832e-06]  MomentsOfInertiaUnits=kg*m^2  ProductsOfInertia=[-1.3611150729646471e-09 1.7933208650124919e-09 9.7887911659441805e-10]  ProductsOfInertiaUnits=kg*m^2  GraphicType=FromGeometry  MarkerShape=Sphere  MarkerSize=10  GraphicVisPropType=SimpleVisualProperties  GraphicDiffuseColor=[0.5 0.5 0.5]  GraphicOpacity=1  GraphicSpecularColor=[0.5 0.5 0.5 1.0]  GraphicAmbientColor=[0.15 0.15 0.15 1.0]  GraphicEmissiveColor=[0.0 0.0 0.0 1.0]  GraphicShininess=75  DoExposeReferenceFrame=on  SerializedFrames=<Frames/>
  Rigid_6_to_8mm_Coupler_v2_1 Placement : sm_lib/Frames and Transforms/Rigid Transform  RotationMethod=RotationMatrix  FollAlignAxisA=+X  BaseAlignAxisA=+Y  FollAlignAxisB=+Y  BaseAlignAxisB=+Z  RotationStandardAxis=+Z  RotationAngle=0  RotationAngleUnits=deg  RotationArbitraryAxis=[0 0 1]  RotationSequenceAxes=FollowerAxes  RotationSequence=XYX  RotationSequenceAngles=[0 0 0]  RotationSequenceAnglesUnits=deg  RotationMatrix=p.parts(5).rotation  Quaternion=[1 0 0 0]  TranslationMethod=Cartesian  TranslationCartesianOffset=p.parts(5).translation  TranslationCartesianOffsetUnits=m  TranslationStandardAxis=+Z  TranslationStandardOffset=0  TranslationStandardOffsetUnits=m  TranslationROffset=0  TranslationROffsetUnits=m  TranslationThetaOffset=0  TranslationThetaOffsetUnits=deg  TranslationZOffset=0  TranslationZOffsetUnits=m
  Solver : nesl_utility/Solver Configuration  PhysicalDomain=network_engine_domain  SubClassName=solver  LeftPortType=input  RightPortType=generic  Tones=[]  Harmonics=[]  SimulateNoise=off  Profile=off  UseLocalSampling=off  EnableSwitchedLinearOptims=on  FrequencyDomain=off  UseCCode=off  RelTol=0.001  AbsTol=0.001  MinStep=1e-09  ToWorkspace=off  RevertToSquareIcSolve=off  NumHomotopyIterations=100  PhasorMode=off  PhasorModeNumHarmonics=1  ConsistencySolver=NEWTON_XTOL_AFTER_FTOL  CanonicalOrdering=CANONICAL  OptimizeIntermediates=OPTIMIZED  MulticoreSolverChoice=BACKWARD_EULER  IndexReductionMethod=DerivativeReplacement  DoDC=off  ResidualTolerance=1e-09  ConsistencyTolSource=GLOBAL  ConsistencyAbsTol=0.001  ConsistencyRelTol=0.001  ConsistencyTolFactor=0.001  UseLocalSolver=off  LocalSolverChoice=NE_BACKWARD_EULER_ADVANCER  ResolveIndetEquations=on  FunctionEvalNumThread=1  LocalSolverSampleTime=0.001  DoFixedCost=off  MaxNonlinIter=3  MaxModeIter=2  ComputeImpulses=off  ImpulseIterations=2  LinearAlgebra=auto  LinearAlgebraNumThread=0  EquationFormulation=NE_TIME_EF  DelaysMemoryBudget=1024  AutomaticFiltering=on  FilteringTimeConstant=0.001  PartitionStorageMethod=AS_NEEDED  PartitionMemoryBudget=1024  PartitionMethod=BALANCED  MultibodyUseLocalSolver=off  MultibodyLocalSolverChoice=ODE1  MultibodyLocalSolverSampleTime=0.001
  State Scope : Scope  NumInputPorts=4
      settings: Title=Arm angle  YLabel=rad
  State Vector : Mux
  Torque Interface : nesl_utility/Simulink-PS Converter  PhysicalDomain=network_engine_domain  SubClassName=ps_input  LeftPortType=input  RightPortType=output  PseudoPeriodic=off  Frequencies=[]  NoiseDistribution=none  NoiseParameters=[]  Unit=N*m  AffineConversion=off  FilteringAndDerivatives=zero  SimscapeFilterOrder=1  InputFilterTimeConstant=0.001  UdotUserProvided=0
  World : sm_lib/Frames and Transforms/World Frame
  motor_holder_1 : sm_lib/Body Elements/File Solid  ExtGeomFileName=D:\university new\Modern Control\project\cad\simscape-exports\motor_holder_1.stl  UnitType=Custom  ExtGeomFileUnits=m  StepReaderType=HEX  ExportConvexHullGeometry=off  InertiaType=Custom  BasedOnType=DensityFromFile  Density=1000  DensityUnits=kg/m^3  Mass=0.0075233994743633126  MassUnits=kg  CenterOfMass=[1.8956047882184069e-14 0.008406159144641271 -0.0085158875958703823]  CenterOfMassUnits=m  MomentsOfInertia=[1.5608911793882638e-06 1.2768019648658448e-06 1.1714557110419128e-06]  MomentsOfInertiaUnits=kg*m^2  ProductsOfInertia=[4.4488416192263043e-07 1.1382738703768502e-18 -1.7963687713376823e-18]  ProductsOfInertiaUnits=kg*m^2  GraphicType=FromGeometry  MarkerShape=Sphere  MarkerSize=10  GraphicVisPropType=SimpleVisualProperties  GraphicDiffuseColor=[0.5 0.5 0.5]  GraphicOpacity=1  GraphicSpecularColor=[0.5 0.5 0.5 1.0]  GraphicAmbientColor=[0.15 0.15 0.15 1.0]  GraphicEmissiveColor=[0.0 0.0 0.0 1.0]  GraphicShininess=75  DoExposeReferenceFrame=on  SerializedFrames=<Frames/>
  motor_holder_1 Placement : sm_lib/Frames and Transforms/Rigid Transform  RotationMethod=RotationMatrix  FollAlignAxisA=+X  BaseAlignAxisA=+Y  FollAlignAxisB=+Y  BaseAlignAxisB=+Z  RotationStandardAxis=+Z  RotationAngle=0  RotationAngleUnits=deg  RotationArbitraryAxis=[0 0 1]  RotationSequenceAxes=FollowerAxes  RotationSequence=XYX  RotationSequenceAngles=[0 0 0]  RotationSequenceAnglesUnits=deg  RotationMatrix=p.parts(2).rotation  Quaternion=[1 0 0 0]  TranslationMethod=Cartesian  TranslationCartesianOffset=p.parts(2).translation  TranslationCartesianOffsetUnits=m  TranslationStandardAxis=+Z  TranslationStandardOffset=0  TranslationStandardOffsetUnits=m  TranslationROffset=0  TranslationROffsetUnits=m  TranslationThetaOffset=0  TranslationThetaOffsetUnits=deg  TranslationZOffset=0  TranslationZOffsetUnits=m
  Angles and Rates : Outport
  Arm Speed rad_s : Outport  Port=2
  wires:
  Drive Torque Nm/1 -> Torque Interface/1
  State Vector/1 -> Angles and Rates/1
  Pendulum Rate rad_s/1 -> State Scope/4, State Vector/4
  Arm Rate rad_s/1 -> State Scope/2, Arm Speed rad_s/1, State Vector/3
  Pendulum Angle rad/1 -> State Scope/3, State Vector/2
  Arm Angle rad/1 -> State Scope/1, State Vector/1
  connections:
  Pendulum Joint/RConn3 -- Pendulum Rate rad_s/LConn1
  Arm Joint/RConn3 -- Arm Rate rad_s/LConn1
  Pendulum Joint/RConn2 -- Pendulum Angle rad/LConn1
  Arm Joint/RConn2 -- Arm Angle rad/LConn1
  Torque Interface/RConn1 -- Arm Joint/LConn2
  Fixed_Profile_2 Placement/RConn1 -- Fixed_Profile_2/RConn1
  Fixed_Profile_1 Placement/RConn1 -- Fixed_Profile_1/RConn1
  ALLEN_04_mm_1 Placement/RConn1 -- ALLEN_04_mm_1/RConn1
  Rigid_6_to_8mm_Coupler_v2_1 Placement/RConn1 -- Rigid_6_to_8mm_Coupler_v2_1/RConn1
  ALLEN_04_mm_1 Placement/LConn1 -- Pendulum Joint/RConn1 -- Rigid_6_to_8mm_Coupler_v2_1 Placement/LConn1
  ROTERY_ENCODER_step_2 Placement/RConn1 -- ROTERY_ENCODER_step_2/RConn1
  Assembly2_1 Placement/RConn1 -- Assembly2_1/RConn1
  motor_holder_1 Placement/RConn1 -- motor_holder_1/RConn1
  Motor_1 Placement/RConn1 -- Motor_1/RConn1
  Pendulum Hinge Frame/RConn1 -- Pendulum Joint/LConn1
  ROTERY_ENCODER_step_2 Placement/LConn1 -- Assembly2_1 Placement/LConn1 -- Reflected Motor and Gear Inertia/RConn1 -- Arm Joint/RConn1 -- Pendulum Hinge Frame/LConn1
  Fixed_Profile_2 Placement/LConn1 -- Fixed_Profile_1 Placement/LConn1 -- motor_holder_1 Placement/LConn1 -- Motor_1 Placement/LConn1 -- Assembly Mounting Frame/RConn1 -- Arm Joint/LConn1
  Assembly Mounting Frame/LConn1 -- Solver/RConn1 -- World/RConn1 -- Gravity/RConn1

== matlab function furuta_hybrid_model/Swing-Up/Torque and Motor Voltage/Inverse Mechanics ==
  data: state input; torque output; acceleration input
function torque = inverse(state,acceleration)
p.L0 = 0.20000000000000001;
p.l1 = 0.14000000000000001;
p.m1 = 0.11;
p.J0 = 0.0070000000000000001;
p.J1cm = 0.001;
p.J1ax = 1.0000000000000001e-05;
p.b0 = 0.0011999999999999999;
p.b1 = 0.00040000000000000002;
p.R = 4;
p.Kt = 0.035000000000000003;
p.Ke = 0.035000000000000003;
p.N = 5;
p.eta = 0.84999999999999998;
p.g = 9.8100000000000005;
torque = furuta_swingup_torque(state,acceleration,p);
end
function torque = furuta_swingup_torque(state,acceleration,p)
% Invert the provisional swing-up plant for the requested arm acceleration.
s = sin(state(2));
c = cos(state(2));
armRate = state(3);
pendulumRate = state(4);
Jp = p.J1cm+p.m1*p.l1^2;
difference = Jp-p.J1ax;
coupling = p.m1*p.L0*p.l1;
targetEnergy = p.m1*p.g*p.l1;
M11 = p.J0+p.m1*p.L0^2+Jp*s^2+p.J1ax*c^2;
M12 = coupling*c;
velocity0 = 2*difference*s*c*armRate*pendulumRate-coupling*s*pendulumRate^2;
pendulumForce = difference*s*c*armRate^2+targetEnergy*s-p.b1*pendulumRate;
pendulumAcceleration = (pendulumForce-M12*acceleration)/Jp;
torque = M11*acceleration+M12*pendulumAcceleration+velocity0+p.b0*armRate;
end
